simulink model "DS_CDMA"  (R2018b)
settings: Solver=VariableStepAuto  StartTime=0.0  StopTime=5  RelTol=1e-3
libraries: commdigbbndpm3 x4, commutil2 x4, commseqgen3 x4, commsink2 x2, simulink x2, commfilt2 x2, commrandsrc3 x2, commchan3 x1
settings Model: Creator=asus  LastModifiedBy=asus

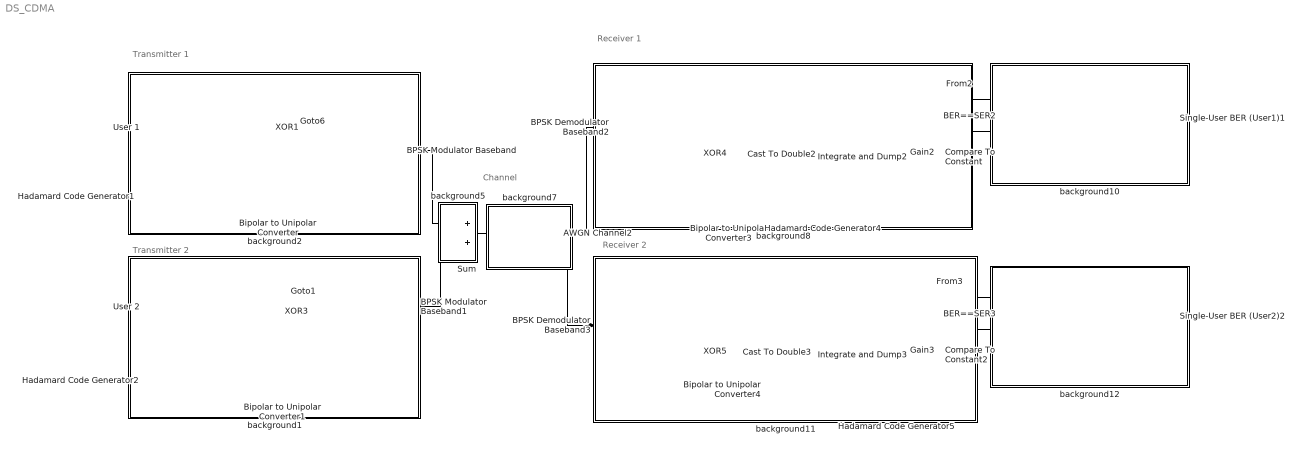
== system DS_CDMA ==
  note: Transmitter 1
  note: Channel
  note: Receiver 2
  note: Transmitter 2
  note: Receiver 1
  AWGN Channel2 : commchan3/AWGN Channel  InputProcessing=Columns as channels (frame based)  seed=1237  noiseMode="Signal to noise ratio  (SNR)"  EbNodB=10  EsNodB=25  SNRdB=5  bitsPerSym=1  Ps=1  Tsym=ts  variance=1
  BER==SER2 : commsink2/Error Rate Calculation  N=0  st_delay=0  cp_mode=Entire frame  subframe=[]  PMode=Port  WsName=ErrorVec  RsMode2=off  stop=off  numErr=100  maxBits=1e6
  BER==SER3 : commsink2/Error Rate Calculation  N=0  st_delay=0  cp_mode=Entire frame  subframe=[]  PMode=Port  WsName=ErrorVec  RsMode2=off  stop=off  numErr=100  maxBits=1e6
  BPSK Demodulator Baseband2 : commdigbbndpm3/BPSK Demodulator Baseband  DecType=Hard decision  VarSource=Dialog  Variance=1  Ph=0  outDtype=Inherit via internal rule  derotateFactorWordLen=16  derotateFactorDataTypeStr=Inherit: Same word length as input  derotateFactorLastDataTypeStr=Inherit: Same word length as input
  BPSK Demodulator Baseband3 : commdigbbndpm3/BPSK Demodulator Baseband  DecType=Hard decision  VarSource=Dialog  Variance=1  Ph=0  outDtype=Inherit via internal rule  derotateFactorWordLen=16  derotateFactorDataTypeStr=Inherit: Same word length as input  derotateFactorLastDataTypeStr=Inherit: Same word length as input
  BPSK Modulator Baseband : commdigbbndpm3/BPSK Modulator Baseband  Ph=0  outDtype=double  outWordLen=16  outUDDataType=sfix(16)  outFracLenMode=Best precision  outFracLen=15  outDataTypeStr=double  outLastDataTypeStr=double
  BPSK Modulator Baseband1 : commdigbbndpm3/BPSK Modulator Baseband  Ph=0  outDtype=double  outWordLen=16  outUDDataType=sfix(16)  outFracLenMode=Best precision  outFracLen=15  outDataTypeStr=double  outLastDataTypeStr=double
  Bipolar to Unipolar Converter{,1,3..4} (4 alike) : commutil2/Bipolar to Unipolar Converter  M=2  polarity=Positive  dataType=Inherit via internal rule
      settings: SourceProductName=Communications System Toolbox  SourceProductBaseCode=CM
  Cast To Double2 : DataTypeConversion  OutDataTypeStr=double
  Cast To Double3 : DataTypeConversion  OutDataTypeStr=double
  Compare To Constant : simulink/Logic and Bit Operations/Compare To Constant  relop=>  const=0.5  OutDataTypeStr=boolean
  Compare To Constant2 : simulink/Logic and Bit Operations/Compare To Constant  relop=>  const=0.5  OutDataTypeStr=boolean
  Gain2 : Gain  Gain=1/8  OutMin=[0]  OutMax=[1]
  Gain3 : Gain  Gain=1/8  OutMin=[0]  OutMax=[1]
  Hadamard Code Generator1 : commseqgen3/Hadamard Code Generator  Length=8  Index=0  SampleTime=1/1000  SamplesPerFrame=8  OutputDataType=double  SimulateUsing=Code generation
      settings: SourceProductName=Communications System Toolbox  SourceProductBaseCode=CM
  Hadamard Code Generator2 : commseqgen3/Hadamard Code Generator  Length=8  Index=5  SampleTime=1/1000  SamplesPerFrame=8  OutputDataType=double  SimulateUsing=Code generation
      settings: SourceProductName=Communications System Toolbox  SourceProductBaseCode=CM
  Hadamard Code Generator4 : commseqgen3/Hadamard Code Generator  Length=8  Index=0  SampleTime=1/1000  SamplesPerFrame=8  OutputDataType=double  SimulateUsing=Code generation
      settings: SourceProductName=Communications System Toolbox  SourceProductBaseCode=CM
  Hadamard Code Generator5 : commseqgen3/Hadamard Code Generator  Length=8  Index=5  SampleTime=1/1000  SamplesPerFrame=8  OutputDataType=double  SimulateUsing=Code generation
      settings: SourceProductName=Communications System Toolbox  SourceProductBaseCode=CM
  Integrate and Dump2 : commfilt2/Integrate and Dump  obssamples=8  offsetsamples=0  nodump=off  roundingMode=Floor  overflowMode=off  outputDataTypeStr=Inherit: Same as accumulator  outputLastDataTypeStr=Inherit: Same as accumulator
  Integrate and Dump3 : commfilt2/Integrate and Dump  obssamples=8  offsetsamples=0  nodump=off  roundingMode=Floor  overflowMode=off  outputDataTypeStr=Inherit: Same as accumulator  outputLastDataTypeStr=Inherit: Same as accumulator
  Single-User BER (User1)1 : Display
  Single-User BER (User2)2 : Display
  Sum : Sum  SaturateOnIntegerOverflow=on
  User 1 : commrandsrc3/Random Integer Generator  SetSize=2  SeedSource=Parameter  Seed=37  SampleTime=1/1000  SamplesPerFrame=1  OutputDataType=boolean  SimulateUsing=Interpreted execution
  User 2 : commrandsrc3/Random Integer Generator  SetSize=2  SeedSource=Parameter  Seed=37  SampleTime=1/1000  SamplesPerFrame=1  OutputDataType=boolean  SimulateUsing=Interpreted execution
  XOR{1,3..5} (4 alike) : Logic  Operator=XOR  IconShape=distinctive  AllPortsSameDT=off  OutDataTypeStr=boolean
  background1 : Subsystem
      mask Display: disp('')
  background10 : Subsystem
      mask Display: disp('')
  background11 : Subsystem
      mask Display: disp('')
  background12 : Subsystem
      mask Display: disp('')
  background2 : Subsystem
      mask Display: disp('')
  background5 : Subsystem
      mask Display: disp('')
  background7 : Subsystem
      mask Display: disp('')
  background8 : Subsystem
      mask Display: disp('')
  tag scope: User1Tx=global, User2Tx=global
  wires:
  User 1/1 -> XOR1/1, [User1Tx]
  XOR1/1 -> BPSK Modulator Baseband/1
  User 2/1 -> [User2Tx], XOR3/1
  XOR3/1 -> BPSK Modulator Baseband1/1
  [User1Tx] -> BER==SER2/1
  Integrate and Dump2/1 -> Gain2/1
  BPSK Demodulator Baseband2/1 -> XOR4/1
  XOR4/1 -> Cast To Double2/1
  BER==SER2/1 -> Single-User BER (User1)1/1
  Cast To Double2/1 -> Integrate and Dump2/1
  [User2Tx] -> BER==SER3/1
  Integrate and Dump3/1 -> Gain3/1
  AWGN Channel2/1 -> BPSK Demodulator Baseband3/1, BPSK Demodulator Baseband2/1
  BPSK Demodulator Baseband3/1 -> XOR5/1
  XOR5/1 -> Cast To Double3/1
  BER==SER3/1 -> Single-User BER (User2)2/1
  Cast To Double3/1 -> Integrate and Dump3/1
  Sum/1 -> AWGN Channel2/1
  BPSK Modulator Baseband1/1 -> Sum/2
  BPSK Modulator Baseband/1 -> Sum/1
  Hadamard Code Generator1/1 -> Bipolar to Unipolar Converter/1
  Bipolar to Unipolar Converter/1 -> XOR1/2
  Hadamard Code Generator2/1 -> Bipolar to Unipolar Converter1/1
  Bipolar to Unipolar Converter1/1 -> XOR3/2
  Hadamard Code Generator4/1 -> Bipolar to Unipolar Converter3/1
  Bipolar to Unipolar Converter3/1 -> XOR4/2
  Bipolar to Unipolar Converter4/1 -> XOR5/2
  Hadamard Code Generator5/1 -> Bipolar to Unipolar Converter4/1
  Compare To Constant/1 -> BER==SER2/2
  Gain3/1 -> Compare To Constant2/1
  Compare To Constant2/1 -> BER==SER3/2
  Gain2/1 -> Compare To Constant/1

== system DS_CDMA/background1 ==

== system DS_CDMA/background10 ==

== system DS_CDMA/background11 ==

== system DS_CDMA/background12 ==

== system DS_CDMA/background2 ==

== system DS_CDMA/background5 ==

== system DS_CDMA/background7 ==

== system DS_CDMA/background8 ==
